simulink model "degrade_with_friction_2dof_two_springs"  (R2025b)
settings: Solver=ode4  StartTime=0.0  StopTime=test_length  FixedStep=step_size  RelTol=1e-3
model workspace (MATLAB code in the model file):
  | starting_k = 1500;
  | stopping_k = 500;
  | step_size = 0.001;
  | test_length = 120;
  | m=1;
  | c=.2;
  | freq = 5;
  | n_tests = 5;
  | 
  | with_friction = true;
  | % friction element
  | F_brk = 0.05;
  | v_brk = 0.01;
  | F_c = 0.9*F_brk;
  | 
  | % time point range of first line segment end (as a ratio of test length)
  | x_range1 = [0.25, 0.45];
  | x_range2 = [0.55, 0.75];
  | % percentage of possible degredation at time point 1 and 2
  | y_range1 = [.57, .85];
  | y_range2 = [.14, .43];
  | %%
  | n_timesteps = floor(test_length/step_size);
  | t = linspace(0, test_length, n_timesteps)';
  | F = sin(2*pi*freq*t);
  | F_signal = [t, F];
  | 
  | x1 = x_range1(1) + rand()*(x_range1(2)-x_range1(1));
  | x2 = x_range2(1) + rand()*(x_range2(2)-x_range2(1));
  | y1 = y_range1(1) + rand()*(y_range1(2)-y_range1(1));
  | y2 = y_range2(1) + rand()*(y_range2(2)-y_range2(1));
  | 
  | y_interp = [1, 1, y1, y2, 0, 0];
  | x_interp = [0, 0.15, x1, x2, 0.85, 1];
  | y_interp = (starting_k - stopping_k)*y_interp + stopping_k;
  | x_interp = x_interp*test_length;
  | 
  | k = interp1(x_interp, y_interp, t);
  | k_signal = [t, k];
values from neighbouring files (symbols this model uses):
  c1 = 0.1    [two_dof_two_springs.m]    (also in twodof_run_experiments.m)
  c2 = 0.2    [two_dof_two_springs.m]    (also in twodof_run_experiments.m)
libraries: fl_lib x13, nesl_utility x10
settings Model: Creator=dncob  LastModifiedBy=cjwil
settings DebuggingCC: UnconnectedInputMsg=warning  UnconnectedOutputMsg=warning  UnconnectedLineMsg=warning
settings ModelReferenceCC: EnableRefExpFcnMdlSchedulingChecks=on
settings RTWCC: GPUComputeCapability=3.5  DLArmComputeVersion=19.05

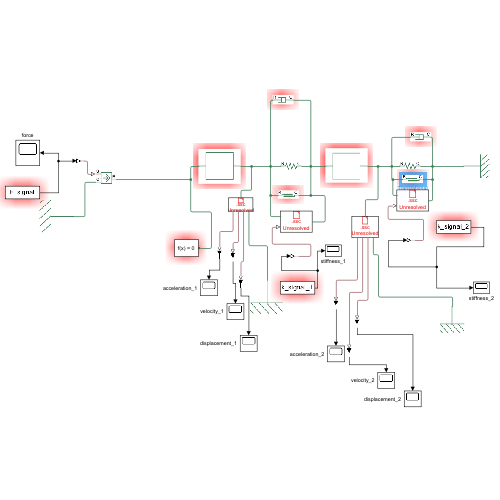
[thumbnail: Simulink's stored preview of the top-level diagram]
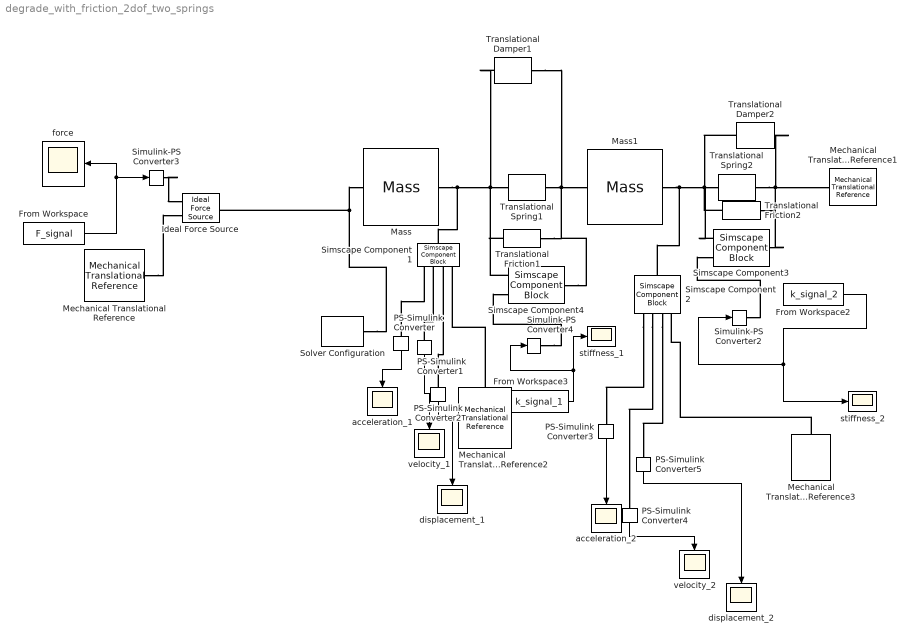
== system degrade_with_friction_2dof_two_springs ==
  From Workspace : FromWorkspace  VariableName=F_signal  SampleTime=step_size  OutputAfterFinalValue=Holding final value
  From Workspace2 : FromWorkspace  VariableName=k_signal_2  SampleTime=step_size  OutputAfterFinalValue=Holding final value
  From Workspace3 : FromWorkspace  VariableName=k_signal_1  SampleTime=step_size  OutputAfterFinalValue=Holding final value
  Ideal Force Source : fl_lib/Mechanical/Mechanical Sources/Ideal Force Source
  Mass : fl_lib/Mechanical/Translational Elements/Mass  mass=m1 kg  num_ports=foundation.enum.numPorts2.two  v_specify=off  v_priority=High  v=0 m/s  v_nominal_specify=off  v_nominal_value=1  v_nominal_unit=m/s  f_specify=off  f_priority=None  f=0 N  f_nominal_specify=off  f_nominal_value=1  f_nominal_unit=N
      settings: InternalSimscapePortConfiguration="{\"Bottom\":[],\"Left\":[{\"id\":\"M\",\"label\":\"\",\"type\":\"foundation.mechanical.translational.translational\"}],\"Right\":[{\"id\":\"N\",\"label\":\"\",\"type\":\"foundation.mechanical.translational.translational\"}],\"Top\":[]}"
  Mass1 : fl_lib/Mechanical/Translational Elements/Mass  mass=m2 kg  num_ports=foundation.enum.numPorts2.two  v_specify=off  v_priority=High  v=0 m/s  v_nominal_specify=off  v_nominal_value=1  v_nominal_unit=m/s  f_specify=off  f_priority=None  f=0 N  f_nominal_specify=off  f_nominal_value=1  f_nominal_unit=N
      settings: InternalSimscapePortConfiguration="{\"Bottom\":[],\"Left\":[{\"id\":\"M\",\"label\":\"\",\"type\":\"foundation.mechanical.translational.translational\"}],\"Right\":[{\"id\":\"N\",\"label\":\"\",\"type\":\"foundation.mechanical.translational.translational\"}],\"Top\":[]}"
  Mechanical Translational Reference{,1..3} (4 alike) : fl_lib/Mechanical/Translational Elements/Mechanical Translational Reference
  PS-Simulink Converter{,1..5} (6 alike) : nesl_utility/PS-Simulink Converter  PhysicalDomain=network_engine_domain  SubClassName=ps_output  LeftPortType=input  RightPortType=output  PseudoPeriodic=off  Frequencies=[]  VectorFormat=inherit  Unit=inherit  AffineConversion=off
  Simscape Component1 : SimscapeComponentBlock  SourceFile=v_a_viewer  ComponentPath=v_a_viewer  ComponentVariants="[\"v_a_viewer\"]"  ComponentVariantNames="[\"v_a_viewer\"]"  ClassName=v_a_viewer  SchemaVersion=1  offset=0 m
      settings: CopyFcn=simscape.sscblock.internal.componentBlockCallback(gcbh,'COPY')  PreCopyFcn=simscape.sscblock.internal.componentBlockCallback(gcbh,'PRECOPY')  PreDeleteFcn=simscape.sscblock.internal.componentBlockCallback(gcbh,'PREDELETE')  InternalSimscapePortConfiguration="{\"Bottom\":[],\"Left\":[{\"id\":\"R\",\"label\":\"R\",\"type\":\"foundation.mechanical.translational.translational\"}],\"Right\":[{\"id\":\"C\",\"label\":\"C\",\"type\":\"foundation.mechanical.translational.translational\"},{\"id\":\"p\",\"label\":\"p\",\"type\":\"output\"},{\"id\":\"v\",\"label\":\"v\",\"type\":\"output\"},{\"id\":\"a\",\"label\":\"a\",\"type\":\"output\"}],\"Top\":[]}"
      mask Type: v_a_viewer
  Simscape Component2 : SimscapeComponentBlock  SourceFile=v_a_viewer  ComponentPath=v_a_viewer  ComponentVariants="[\"v_a_viewer\"]"  ComponentVariantNames="[\"v_a_viewer\"]"  ClassName=v_a_viewer  SchemaVersion=1  offset=0 m
      settings: CopyFcn=simscape.sscblock.internal.componentBlockCallback(gcbh,'COPY')  PreCopyFcn=simscape.sscblock.internal.componentBlockCallback(gcbh,'PRECOPY')  PreDeleteFcn=simscape.sscblock.internal.componentBlockCallback(gcbh,'PREDELETE')  InternalSimscapePortConfiguration="{\"Bottom\":[],\"Left\":[{\"id\":\"R\",\"label\":\"R\",\"type\":\"foundation.mechanical.translational.translational\"}],\"Right\":[{\"id\":\"C\",\"label\":\"C\",\"type\":\"foundation.mechanical.translational.translational\"},{\"id\":\"p\",\"label\":\"p\",\"type\":\"output\"},{\"id\":\"v\",\"label\":\"v\",\"type\":\"output\"},{\"id\":\"a\",\"label\":\"a\",\"type\":\"output\"}],\"Top\":[]}"
      mask Type: v_a_viewer
  Simscape Component3 : SimscapeComponentBlock  SourceFile=time_variable_spring  ComponentPath=time_variable_spring  ComponentVariants="[\"time_variable_spring\"]"  ComponentVariantNames="[\"time_variable_spring\"]"  ClassName=time_variable_spring  SchemaVersion=1  v_specify=off  v_priority=None  v=0 m/s  v_nominal_specify=off  v_nominal_value=1  v_nominal_unit=m/s  f_specify=off  f_priority=None  f=0 N  f_nominal_specify=off  f_nominal_value=1  f_nominal_unit=N  x_specify=off  x_priority=High  x=0 m  x_nominal_specify=off  x_nominal_value=1  x_nominal_unit=m
      settings: CopyFcn=simscape.sscblock.internal.componentBlockCallback(gcbh,'COPY')  PreCopyFcn=simscape.sscblock.internal.componentBlockCallback(gcbh,'PRECOPY')  PreDeleteFcn=simscape.sscblock.internal.componentBlockCallback(gcbh,'PREDELETE')  InternalSimscapePortConfiguration="{\"Bottom\":[],\"Left\":[{\"id\":\"R\",\"label\":\"R\",\"type\":\"foundation.mechanical.translational.translational\"},{\"id\":\"k\",\"label\":\"k\",\"type\":\"input\"}],\"Right\":[{\"id\":\"C\",\"label\":\"C\",\"type\":\"foundation.mechanical.translational.translational\"}],\"Top\":[]}"
      mask Type: Translational Spring
  Simscape Component4 : SimscapeComponentBlock  SourceFile=time_variable_spring  ComponentPath=time_variable_spring  ComponentVariants="[\"time_variable_spring\"]"  ComponentVariantNames="[\"time_variable_spring\"]"  ClassName=time_variable_spring  SchemaVersion=1  v_specify=off  v_priority=None  v=0 m/s  v_nominal_specify=off  v_nominal_value=1  v_nominal_unit=m/s  f_specify=off  f_priority=None  f=0 N  f_nominal_specify=off  f_nominal_value=1  f_nominal_unit=N  x_specify=off  x_priority=High  x=0 m  x_nominal_specify=off  x_nominal_value=1  x_nominal_unit=m
      settings: CopyFcn=simscape.sscblock.internal.componentBlockCallback(gcbh,'COPY')  PreCopyFcn=simscape.sscblock.internal.componentBlockCallback(gcbh,'PRECOPY')  PreDeleteFcn=simscape.sscblock.internal.componentBlockCallback(gcbh,'PREDELETE')  InternalSimscapePortConfiguration="{\"Bottom\":[],\"Left\":[{\"id\":\"R\",\"label\":\"R\",\"type\":\"foundation.mechanical.translational.translational\"},{\"id\":\"k\",\"label\":\"k\",\"type\":\"input\"}],\"Right\":[{\"id\":\"C\",\"label\":\"C\",\"type\":\"foundation.mechanical.translational.translational\"}],\"Top\":[]}"
      mask Type: Translational Spring
  Simulink-PS Converter2 : nesl_utility/Simulink-PS Converter  PhysicalDomain=network_engine_domain  SubClassName=ps_input  LeftPortType=input  RightPortType=output  PseudoPeriodic=off  Frequencies=[]  NoiseDistribution=none  NoiseParameters=[]  Unit=1  AffineConversion=off  FilteringAndDerivatives=provide  SimscapeFilterOrder=1  InputFilterTimeConstant=0.001  UdotUserProvided=0
  Simulink-PS Converter3 : nesl_utility/Simulink-PS Converter  PhysicalDomain=network_engine_domain  SubClassName=ps_input  LeftPortType=input  RightPortType=output  PseudoPeriodic=off  Frequencies=[]  NoiseDistribution=none  NoiseParameters=[]  Unit=1  AffineConversion=off  FilteringAndDerivatives=provide  SimscapeFilterOrder=1  InputFilterTimeConstant=0.001  UdotUserProvided=0
  Simulink-PS Converter4 : nesl_utility/Simulink-PS Converter  PhysicalDomain=network_engine_domain  SubClassName=ps_input  LeftPortType=input  RightPortType=output  PseudoPeriodic=off  Frequencies=[]  NoiseDistribution=none  NoiseParameters=[]  Unit=1  AffineConversion=off  FilteringAndDerivatives=provide  SimscapeFilterOrder=1  InputFilterTimeConstant=0.001  UdotUserProvided=0
  Solver Configuration : nesl_utility/Solver Configuration  PhysicalDomain=network_engine_domain  SubClassName=solver  LeftPortType=input  RightPortType=generic  Tones=[]  Harmonics=[]  SimulateNoise=off  Profile=off  UseLocalSampling=off  EnableSwitchedLinearOptims=on  FrequencyDomain=off  UseCCode=off  RelTol=0.001  AbsTol=0.001  MinStep=1e-09  ToWorkspace=off  RevertToSquareIcSolve=off  NumHomotopyIterations=100  PhasorMode=off  PhasorModeNumHarmonics=1  ConsistencySolver=NEWTON_XTOL_AFTER_FTOL  IndexReductionMethod=DerivativeReplacement  DoDC=off  ResidualTolerance=1e-09  ConsistencyTolSource=GLOBAL  ConsistencyAbsTol=0.001  ConsistencyRelTol=0.001  ConsistencyTolFactor=0.001  UseLocalSolver=on  LocalSolverChoice=NE_TRAPEZOIDAL_ADVANCER  ResolveIndetEquations=on  FunctionEvalNumThread=1  LocalSolverSampleTime=step_size  DoFixedCost=off  MaxNonlinIter=3  MaxModeIter=2  ComputeImpulses=off  ImpulseIterations=2  LinearAlgebra=auto  LinearAlgebraNumThread=0  EquationFormulation=NE_TIME_EF  DelaysMemoryBudget=1024  AutomaticFiltering=on  FilteringTimeConstant=0.001  PartitionStorageMethod=AS_NEEDED  PartitionMemoryBudget=1024  PartitionMethod=ROBUST  MultibodyUseLocalSolver=off  MultibodyLocalSolverChoice=ODE1  MultibodyLocalSolverSampleTime=0.001
  Translational Friction1 : fl_lib/Mechanical/Translational Elements/Translational Friction  brkwy_frc=F_brk N  brkwy_vel=v_brk m/s  Col_frc=F_c N  visc_coef=0 N*s/m  v_specify=off  v_priority=None  v=0 m/s  v_nominal_specify=off  v_nominal_value=1  v_nominal_unit=m/s  f_specify=off  f_priority=None  f=0 N  f_nominal_specify=off  f_nominal_value=1  f_nominal_unit=N
      settings: InternalSimscapePortConfiguration="{\"Bottom\":[],\"Left\":[{\"id\":\"R\",\"label\":\"R\",\"type\":\"foundation.mechanical.translational.translational\"}],\"Right\":[{\"id\":\"C\",\"label\":\"C\",\"type\":\"foundation.mechanical.translational.translational\"}],\"Top\":[]}"
  Translational Friction2 : fl_lib/Mechanical/Translational Elements/Translational Friction  brkwy_frc=F_brk N  brkwy_vel=v_brk m/s  Col_frc=F_c N  visc_coef=0 N*s/m  v_specify=off  v_priority=None  v=0 m/s  v_nominal_specify=off  v_nominal_value=1  v_nominal_unit=m/s  f_specify=off  f_priority=None  f=0 N  f_nominal_specify=off  f_nominal_value=1  f_nominal_unit=N
      settings: InternalSimscapePortConfiguration="{\"Bottom\":[],\"Left\":[{\"id\":\"R\",\"label\":\"R\",\"type\":\"foundation.mechanical.translational.translational\"}],\"Right\":[{\"id\":\"C\",\"label\":\"C\",\"type\":\"foundation.mechanical.translational.translational\"}],\"Top\":[]}"
  Translational Damper1 : fl_lib/Mechanical/Translational Elements/Translational Damper  D=c1 N*s/m  v_specify=off  v_priority=None  v=0 m/s  v_nominal_specify=off  v_nominal_value=1  v_nominal_unit=m/s  f_specify=off  f_priority=None  f=0 N  f_nominal_specify=off  f_nominal_value=1  f_nominal_unit=N
  Translational Damper2 : fl_lib/Mechanical/Translational Elements/Translational Damper  D=c2 N*s/m  v_specify=off  v_priority=None  v=0 m/s  v_nominal_specify=off  v_nominal_value=1  v_nominal_unit=m/s  f_specify=off  f_priority=None  f=0 N  f_nominal_specify=off  f_nominal_value=1  f_nominal_unit=N
  Translational Spring1 : fl_lib/Mechanical/Translational Elements/Translational Spring  spr_rate=10 N/m  v_specify=off  v_priority=None  v=0 m/s  v_nominal_specify=off  v_nominal_value=1  v_nominal_unit=m/s  f_specify=off  f_priority=None  f=0 N  f_nominal_specify=off  f_nominal_value=1  f_nominal_unit=N  x_specify=off  x_priority=High  x=0 m  x_nominal_specify=off  x_nominal_value=1  x_nominal_unit=m
  Translational Spring2 : fl_lib/Mechanical/Translational Elements/Translational Spring  spr_rate=10 N/m  v_specify=off  v_priority=None  v=0 m/s  v_nominal_specify=off  v_nominal_value=1  v_nominal_unit=m/s  f_specify=off  f_priority=None  f=0 N  f_nominal_specify=off  f_nominal_value=1  f_nominal_unit=N  x_specify=off  x_priority=High  x=0 m  x_nominal_specify=off  x_nominal_value=1  x_nominal_unit=m
  acceleration_1 : Scope
      settings: ActiveDisplayYMinimum=-3.255047314570287  ActiveDisplayYMaximum=3.5539756124055968  DataLoggingVariableName=acceleration_1  DataLoggingSaveFormat=Array
  acceleration_2 : Scope
      settings: ActiveDisplayYMinimum=-1  ActiveDisplayYMaximum=1  DataLoggingVariableName=acceleration_2  DataLoggingSaveFormat=Array
  displacement_1 : Scope
      settings: ActiveDisplayYMinimum=-1  ActiveDisplayYMaximum=1  DataLoggingVariableName=displacement_1  DataLoggingSaveFormat=Array
  displacement_2 : Scope
      settings: ActiveDisplayYMinimum=-1  ActiveDisplayYMaximum=1  DataLoggingVariableName=displacement_2  DataLoggingSaveFormat=Array
  force : Scope
      settings: ActiveDisplayYMinimum=0.03576  ActiveDisplayYMaximum=0.59959  DataLoggingVariableName=force  DataLoggingSaveFormat=Array
  stiffness_1 : Scope
      settings: ActiveDisplayYMinimum=375.21822  ActiveDisplayYMaximum=1624.97575  DataLoggingVariableName=stiffness_1  DataLoggingSaveFormat=Array
  stiffness_2 : Scope
      settings: ActiveDisplayYMinimum=375.21822  ActiveDisplayYMaximum=1624.97575  DataLoggingVariableName=stiffness_2  DataLoggingSaveFormat=Array
  velocity_1 : Scope
      settings: ActiveDisplayYMinimum=-1  ActiveDisplayYMaximum=1  DataLoggingVariableName=velocity_1  DataLoggingSaveFormat=Array
  velocity_2 : Scope
      settings: ActiveDisplayYMinimum=-1  ActiveDisplayYMaximum=1  DataLoggingVariableName=velocity_2  DataLoggingSaveFormat=Array
  wires:
  PS-Simulink Converter1/1 -> velocity_1/1
  PS-Simulink Converter2/1 -> displacement_1/1
  PS-Simulink Converter/1 -> acceleration_1/1
  PS-Simulink Converter3/1 -> acceleration_2/1
  PS-Simulink Converter4/1 -> velocity_2/1
  PS-Simulink Converter5/1 -> displacement_2/1
  From Workspace/1 -> force/1, Simulink-PS Converter3/1
  From Workspace2/1 -> stiffness_2/1, Simulink-PS Converter2/1
  From Workspace3/1 -> stiffness_1/1, Simulink-PS Converter4/1
  connections:
  Solver Configuration/RConn1 -- Mass/RConn1 -- Ideal Force Source/LConn1
  Mass/LConn1 -- Simscape Component4/LConn1 -- Translational Friction1/LConn1 -- Translational Spring1/LConn1 -- Translational Damper1/LConn1 -- Simscape Component1/LConn1
  Translational Spring1/RConn1 -- Simscape Component4/RConn1 -- Translational Friction1/RConn1 -- Translational Damper1/RConn1 -- Mass1/LConn1
  Mass1/RConn1 -- Simscape Component3/LConn1 -- Translational Friction2/LConn1 -- Translational Spring2/LConn1 -- Translational Damper2/LConn1 -- Simscape Component2/LConn1
  Translational Spring2/RConn1 -- Simscape Component3/RConn1 -- Translational Friction2/RConn1 -- Mechanical Translational Reference1/LConn1 -- Translational Damper2/RConn1
  Mechanical Translational Reference2/LConn1 -- Simscape Component1/RConn1
  PS-Simulink Converter/LConn1 -- Simscape Component1/RConn4
  PS-Simulink Converter1/LConn1 -- Simscape Component1/RConn3
  PS-Simulink Converter2/LConn1 -- Simscape Component1/RConn2
  Mechanical Translational Reference3/LConn1 -- Simscape Component2/RConn1
  Simscape Component2/RConn4 -- PS-Simulink Converter3/LConn1
  Simscape Component2/RConn3 -- PS-Simulink Converter4/LConn1
  Simscape Component2/RConn2 -- PS-Simulink Converter5/LConn1
  Mechanical Translational Reference/LConn1 -- Ideal Force Source/RConn2
  Simulink-PS Converter3/RConn1 -- Ideal Force Source/RConn1
  Simulink-PS Converter2/RConn1 -- Simscape Component3/LConn2
  Simulink-PS Converter4/RConn1 -- Simscape Component4/LConn2
